simulink model "elp_hw_frontend"  (R2026b)
settings: Solver=VariableStepAuto
undefined symbols (not defined in the file or in its folder): P, Ts
libraries: simulink x1
settings Model: Creator=aomar  LastModifiedBy=aomar

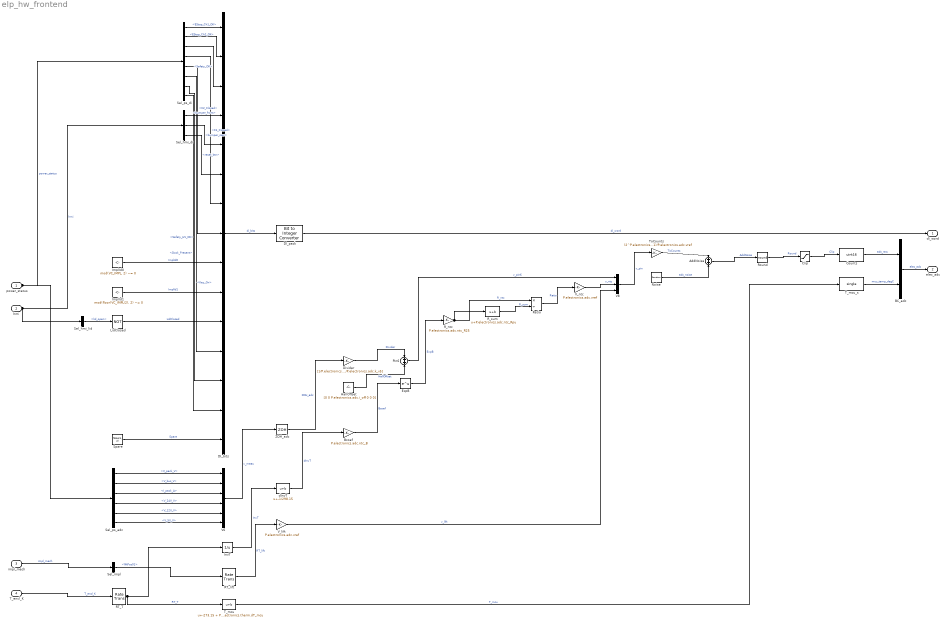
== system elp_hw_frontend ==
  power_status : Inport  OutDataTypeStr=Bus: Bus_PowerStatus  SampleTime=Ts.base
  hmi : Inport  Port=2  OutDataTypeStr=Bus: Bus_HmiInputs  SampleTime=Ts.base
  impl_mech : Inport  Port=3  OutDataTypeStr=Bus: Bus_ImplMechState  SampleTime=Ts.ctrl
  T_encl_K : Inport  Port=4  OutDataTypeStr=double  SampleTime=Ts.hk
  AddNoise : Sum
  BC_adc : BusCreator  Inputs=2  OutDataTypeStr=Bus: Bus_ElecAdc  NonVirtualBus=on
      settings: InheritFromInputs=off
  Bcoef : Gain  Gain=P.electronics.adc.ntc_B
  Clip : Saturate  UpperLimit=2^P.electronics.adc.nbits - 1  LowerLimit=0
  Counts : DataTypeConversion  OutDataTypeStr=uint16  RndMeth=Nearest
  DI_bits : Concatenate  NumInputs=15
  DI_pack : simulink/Logic and Bit Operations/Bit to Integer Converter  nbits=16  bitOrder=LSB first  signedOutputValues=Unsigned  outDtype=uint16  outDtypeSigned=Inherit via internal rule
      settings: LibrarySourceBlock=|
      | commutil2/Bit to Integer
      | Converter
  Divider : Gain  Gain=[1/P.electronics.adc.k_vpack 1/P.electronics.adc.k_vlink P.electronics.adc.i_sens 1/P.electronics.adc.k_v24 1/P.electronics.adc.k_v12 1/P.electronics.adc.k_v5]
  ExpB : Math
  HallOffset : Constant  Value=[0 0 P.electronics.adc.i_off 0 0 0]  OutDataTypeStr=double  SampleTime=Ts.comm
  ImplId0 : Constant  Value=mod(VC_IMPL, 2) ~= 0  OutDataTypeStr=boolean  SampleTime=Ts.base
  ImplId1 : Constant  Value=mod(floor(VC_IMPL/2), 2) ~= 0  OutDataTypeStr=boolean  SampleTime=Ts.base
  InvT : Math  Operator=reciprocal
  LidClosed : Logic  Operator=NOT  Inputs=1  AllPortsSameDT=off  OutDataTypeStr=boolean
  Noise : RandomNumber  Mean=zeros(1, 8)  Variance=P.electronics.adc.noise_lsb^2  Seed=P.electronics.adc.seed + (1:8)  SampleTime=Ts.comm
  Pin6 : Sum
  RT_T : RateTransition  InitialCondition=P.electronics.therm.T0  OutPortSampleTime=Ts.comm
  RT_lift : RateTransition  OutPortSampleTime=Ts.comm
  R_ntc : Gain  Gain=P.electronics.adc.ntc_R25
  R_sum : Bias  Bias=P.electronics.adc.ntc_Rpu  SaturateOnIntegerOverflow=off
  Ratio : Product  Inputs=*/
  Round : Rounding  Operator=round
  Sel_hmi_di : BusSelector  OutputSignals=bumper_front,bumper_rear,reset_btn
  Sel_hmi_lid : BusSelector  OutputSignals=lid_open
  Sel_impl : BusSelector  OutputSignals=liftPos01
  Sel_ps_adc : BusSelector  OutputSignals=V_pack_V,V_bus_V,I_pack_A,V_24V_V,V_12V_V,V_5V_V
  Sel_ps_di : BusSelector  OutputSignals=EStop_Ch1_OK,EStop_Ch2_OK,Safety_OK,K1_Closed,K2_Closed,Key_On,Safety_HV_OK,Dock_Present
  Spare : Constant  Value=false(1, 2)  OutDataTypeStr=boolean  SampleTime=Ts.base
  T_mcu : Bias  Bias=-273.15 + P.electronics.therm.dT_mcu  SaturateOnIntegerOverflow=off
  T_mcu_s : DataTypeConversion  OutDataTypeStr=single  RndMeth=Nearest
  ToCounts : Gain  Gain=(2^P.electronics.adc.nbits - 1)/P.electronics.adc.vref
  V6 : Concatenate  NumInputs=6
  V8 : Concatenate  NumInputs=3
  V_lift : Gain  Gain=P.electronics.adc.vref
  V_ntc : Gain  Gain=P.electronics.adc.vref
  ZOH_adc : ZeroOrderHold  SampleTime=Ts.comm
  dInvT : Bias  Bias=-1/298.15  SaturateOnIntegerOverflow=off
  di_word : Outport  OutDataTypeStr=uint16
  elec_adc : Outport  Port=2  OutDataTypeStr=Bus: Bus_ElecAdc
  wires:
  power_status/1 -> Sel_ps_di/1, Sel_ps_adc/1  "power_status"
  hmi/1 -> Sel_hmi_di/1, Sel_hmi_lid/1  "hmi"
  impl_mech/1 -> Sel_impl/1  "impl_mech"
  T_encl_K/1 -> RT_T/1  "T_encl_K"
  Sel_hmi_lid/1 -> LidClosed/1  "<lid_open>"
  Sel_ps_adc/1 -> V6/1  "<V_pack_V>"
  Sel_ps_adc/2 -> V6/2  "<V_bus_V>"
  Sel_ps_adc/3 -> V6/3  "<I_pack_A>"
  Sel_ps_adc/4 -> V6/4  "<V_24V_V>"
  Sel_ps_adc/5 -> V6/5  "<V_12V_V>"
  Sel_ps_adc/6 -> V6/6  "<V_5V_V>"
  Sel_impl/1 -> RT_lift/1  "<liftPos01>"
  ImplId0/1 -> DI_bits/9  "ImplId0"
  ImplId1/1 -> DI_bits/10  "ImplId1"
  LidClosed/1 -> DI_bits/11  "LidClosed"
  Spare/1 -> DI_bits/15  "Spare"
  RT_T/1 -> InvT/1, T_mcu/1  "RT_T"
  Sel_ps_di/1 -> DI_bits/1  "<EStop_Ch1_OK>"
  Sel_ps_di/2 -> DI_bits/2  "<EStop_Ch2_OK>"
  Sel_ps_di/3 -> DI_bits/3  "<Safety_OK>"
  Sel_ps_di/4 -> DI_bits/7  "<K1_Closed>"
  Sel_ps_di/5 -> DI_bits/8  "<K2_Closed>"
  Sel_ps_di/6 -> DI_bits/12  "<Key_On>"
  Sel_ps_di/7 -> DI_bits/13  "<Safety_HV_OK>"
  Sel_ps_di/8 -> DI_bits/14  "<Dock_Present>"
  Sel_hmi_di/1 -> DI_bits/4  "<bumper_front>"
  Sel_hmi_di/2 -> DI_bits/5  "<bumper_rear>"
  Sel_hmi_di/3 -> DI_bits/6  "<reset_btn>"
  DI_bits/1 -> DI_pack/1  "di_bits"
  V6/1 -> ZOH_adc/1  "v_meas"
  InvT/1 -> dInvT/1  "InvT"
  RT_lift/1 -> V_lift/1  "RT_lift"
  T_mcu/1 -> T_mcu_s/1  "T_mcu"
  V_lift/1 -> V8/3  "v_lift"
  ZOH_adc/1 -> Divider/1  "ZOH_adc"
  dInvT/1 -> Bcoef/1  "dInvT"
  DI_pack/1 -> di_word/1  "di_word"
  Divider/1 -> Pin6/1  "Divider"
  HallOffset/1 -> Pin6/2  "HallOffset"
  Bcoef/1 -> ExpB/1  "Bcoef"
  Pin6/1 -> V8/1  "v_pin6"
  ExpB/1 -> R_ntc/1  "ExpB"
  R_ntc/1 -> Ratio/1, R_sum/1  "R_ntc"
  R_sum/1 -> Ratio/2  "R_sum"
  Ratio/1 -> V_ntc/1  "Ratio"
  V_ntc/1 -> V8/2  "v_ntc"
  V8/1 -> ToCounts/1  "v_pin"
  ToCounts/1 -> AddNoise/1  "ToCounts"
  Noise/1 -> AddNoise/2  "adc_noise"
  AddNoise/1 -> Round/1  "AddNoise"
  Round/1 -> Clip/1  "Round"
  Clip/1 -> Counts/1  "Clip"
  Counts/1 -> BC_adc/1  "adc_raw"
  T_mcu_s/1 -> BC_adc/2  "mcu_temp_degC"
  BC_adc/1 -> elec_adc/1  "elec_adc"
